simulink model "PID"  (R2024b)
settings: Solver=FixedStepAuto  StartTime=0.0  StopTime=inf  FixedStep=0.001  RelTol=1e-3  EnableMultiTasking=on
libraries: slpidlib x1, px4Peripheralslib x1, px4Sensorslib x1
settings Model: SimulationMode=external  ExtModeTrigDuration=10  Creator=ArriGE66  LastModifiedBy=xippa
settings SolverCC: PositivePriorityOrder=on
settings OptimizationCC: EnhancedBackFolding=on  PassReuseOutputArgsAs=Individual arguments  ZeroExternalMemoryAtStartup=off  ZeroInternalMemoryAtStartup=off  MaxStackSize=64  OptimizeBlockOrder=speed  DifferentSizesBufferReuse=on  OptimizationCustomize=off  EfficientTunableParamExpr=on
settings DebuggingCC: ParameterTunabilityLossMsg=error
settings HardwareCC: ProdBitPerPointer=32  ProdBitPerSizeT=32  ProdBitPerPtrDiffT=32  ProdLargestAtomicInteger=Long  ProdLargestAtomicFloat=Double  ProdWordSize=32  ProdLongLongMode=on  ProdHWDeviceType=ARM Compatible->ARM Cortex
settings SFSimCC: MATLABDynamicMemAlloc=off  SimTargetLang=C++
settings RTWCC: Description=Embedded Coder  SystemTargetFile=ert.tlc  HardwareBoard=PX4 Cube Orange  TemplateMakefile=ert_default_tmf  Toolchain=GNU Tools for PX4 Autopilots  TargetLang=C++  GPUComputeCapability=3.5
settings CodeAppCC: ForceParamTrailComments=on  IgnoreCustomStorageClasses=off  OperatorAnnotations=on  SimulinkDataObjDesc=on  SFDataObjDesc=on  InsertBlockDesc=on
settings ERTTargetCC: SupportVariableSizeSignals=on  ExtMode=on  ExtModeTransport=3  ExtModeStaticAlloc=on  ExtModeStaticAllocSize=1024  ExtModeMexFile=ext_xcp  ExtModeMexArgs=1 COM10 3000000  ExtModeIntrfLevel=Level2 - Open  InlinedParameterPlacement=Hierarchical  DynamicArrayContainerType=coder::array

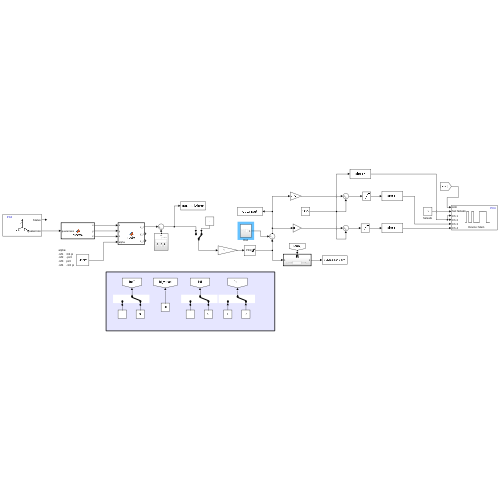
[thumbnail: Simulink's stored preview of the top-level diagram]
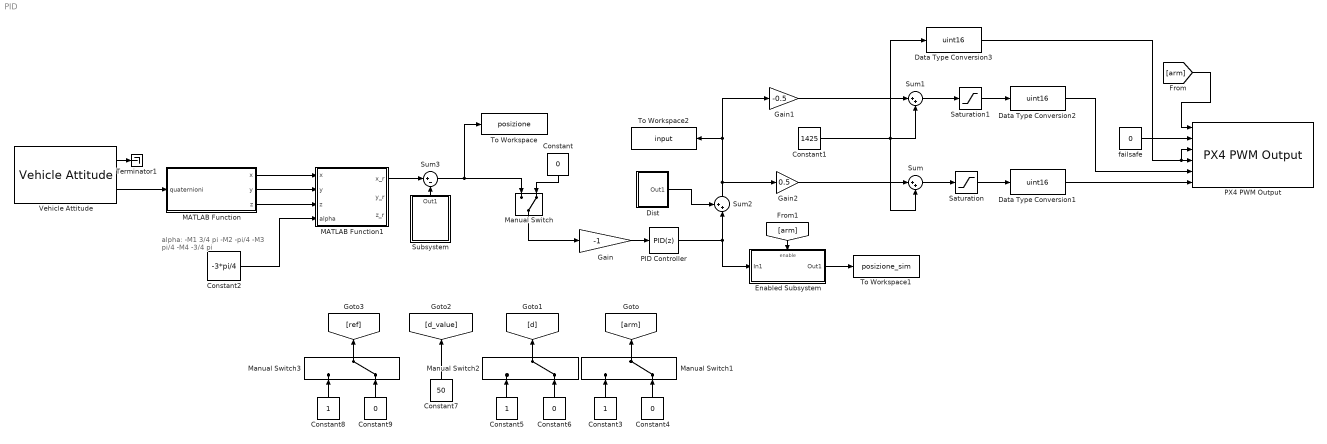
== system PID ==
  note: alpha:
      | -M1    3/4 pi
      | -M2    -pi/4
      | -M3    pi/4
      | -M4    -3/4 pi
  Constant{,4,6,9} (4 alike) : Constant  Value=0
  Constant1 : Constant  Value=1425  SampleTime=0.01
  Constant2 : Constant  Value=-3*pi/4  SampleTime=0.01
  Constant3 : Constant
  Constant5 : Constant
  Constant7 : Constant  Value=50
  Constant8 : Constant
  Data Type Conversion1 : DataTypeConversion  OutDataTypeStr=uint16  SaturateOnIntegerOverflow=off  RndMeth=Floor
  Data Type Conversion2 : DataTypeConversion  OutDataTypeStr=uint16  SaturateOnIntegerOverflow=off  RndMeth=Floor
  Data Type Conversion3 : DataTypeConversion  OutDataTypeStr=uint16  SaturateOnIntegerOverflow=off  RndMeth=Floor
  Dist : Subsystem
  Enabled Subsystem : Subsystem  TreatAsAtomicUnit=on
  Gain : Gain  Gain=-1
  Gain1 : Gain  Gain=-0.5
  Gain2 : Gain  Gain=0.5
  MATLAB Function : MATLAB Function  TreatAsAtomicUnit=on
  MATLAB Function1 : MATLAB Function  TreatAsAtomicUnit=on
  Manual Switch{,1..3} (4 alike) : ManualSwitch  CurrentSetting=0
  PID Controller : slpidlib/PID Controller  Controller=PID  Form=Parallel  TimeDomain=Discrete-time  UseExternalTs=off  SampleTime=-1  IntegratorMethod=Forward Euler  FilterMethod=Forward Euler  ControllerParametersSource=internal  P=400  I=500  UseKiTs=off  D=50  UseExternalDerivativeSource=off  N=880  UseFilter=on  TunerSelectOption=Transfer Function Based (PID Tuner App)  InitialConditionSource=internal  InitialConditionForIntegrator=0  InitialConditionForFilter=0  DifferentiatorICPrevScaledInput=0  ExternalReset=none  TrackingMode=off  Kt=1  LimitOutput=on  SatLimitsSource=internal  UpperSaturationLimit=600  LowerSaturationLimit=-600  LinearizeAsGain=on  AntiWindupMode=clamping  Kb=1  LimitIntegrator=off  UpperIntegratorSaturationLimit=inf  LowerIntegratorSaturationLimit=-inf  POutMin=[]  POutMax=[]  IOutMin=[]  IOutMax=[]  DOutMin=[]  DOutMax=[]  NOutMin=[]  NOutMax=[]  SumOutMin=[]  SumOutMax=[]  SaturationOutMin=[]  SaturationOutMax=[]  PParamMin=[]  PParamMax=[]  IParamMin=[]  IParamMax=[]  DParamMin=[]  DParamMax=[]  NParamMin=[]  NParamMax=[]  KbParamMin=[]  KbParamMax=[]  KtParamMin=[]  KtParamMax=[]  KbOutMin=[]  KbOutMax=[]  KtOutMin=[]  KtOutMax=[]  IntegratorOutMin=[]  IntegratorOutMax=[]  FilterOutMin=[]  FilterOutMax=[]  SumI1OutMin=[]  SumI1OutMax=[]  SumI2OutMin=[]  SumI2OutMax=[]  SumI3OutMin=[]  SumI3OutMax=[]  SumI4OutMin=[]  SumI4OutMax=[]  SumDOutMin=[]  SumDOutMax=[]  DifferentiatorOutMin=[]  DifferentiatorOutMax=[]  FilterDiffOutCoefMin=[]  FilterDiffOutCoefMax=[]  ReciprocalOutMin=[]  ReciprocalOutMax=[]  SumDenOutMin=[]  SumDenOutMax=[]  SumNumOutMin=[]  SumNumOutMax=[]  DivideOutMin=[]  DivideOutMax=[]  UdiffTsProdOutMin=[]  UdiffTsProdOutMax=[]  NTsProdOutMin=[]  NTsProdOutMax=[]  UintegralTsProdOutMin=[]  UintegralTsProdOutMax=[]  UngainTsProdOutMin=[]  UngainTsProdOutMax=[]  ClampingZeroOutDataTypeStr=Inherit: Inherit via back propagation  ClampingZeroOutMin=[]  ClampingZeroOutMax=[]  FilterDenConstantOutDataTypeStr=Inherit: Inherit via back propagation  FilterDenConstantOutMin=[]  FilterDenConstantOutMax=[]  PCopyOutDataTypeStr=Inherit: Inherit via back propagation  PCopyOutMin=[]  PCopyOutMax=[]  NCopyOutDataTypeStr=Inherit: Inherit via back propagation  NCopyOutMin=[]  NCopyOutMax=[]  IntegratorContinuousStateAttributes=''  IntegratorStateMustResolveToSignalObject=off  IntegratorRTWStateStorageClass=Auto  FilterContinuousStateAttributes=''  FilterStateMustResolveToSignalObject=off  FilterRTWStateStorageClass=Auto  ParallelPVariant=InternalParameters  IdealPVariant=Disabled  IVariant=InternalParameters  DVariant=InternalParameters  IntegratorVariant=Discrete  SatVariant=Enabled  AWVariant=DiscClampingParallel  PCopyVariant=Disabled  TRVariant=Disabled  FdbkBlocksVariant=Forward  IdealPFdbkVariant=Disabled  SatFdbkVariant=Disabled  DerivativeFilterVariant=ForwardEulerFilter  NVariant=InternalParameters  NCopyVariant=Disabled  FilterICVariant=InternalICsFilter  IntegratorICVariant=InternalICs  ExternalResetVariant=Disabled  TRSumVariant=Passthrough  SumFdbkVariant=Disabled  SumVariant=Sum_PID  TsampFilterVariant=InternalTs  TsampNgainVariant=Passthrough  TsampIntegralVariant=Disabled_SignalSpec  ExternalSaturationOutDataTypeStr=Inherit: Same as second input  DerivativeSourceVariant=ErrorSignal  PreIntVariant=InternalPreInt
  PX4 PWM Output : px4Peripheralslib/PX4 PWM Output  pwmDevice=Main  pwmChannel1_=on  pwmChannel2_=on  pwmChannel3_=on  pwmChannel4_=on  pwmChannel5_=off  pwmChannel6_=off  pwmChannel7_=off  pwmChannel8_=off
  Saturation : Saturate  UpperLimit=1750  LowerLimit=1050
  Saturation1 : Saturate  UpperLimit=1750  LowerLimit=1050
  Subsystem : Subsystem
  Sum : Sum  Inputs=|++
  Sum1 : Sum  Inputs=|++
  Sum2 : Sum  Inputs=++|
  Sum3 : Sum  Inputs=|+-
  Terminator1 : Terminator
  To Workspace : ToWorkspace  VariableName=posizione  SaveFormat=Timeseries  SampleTime=-1
  To Workspace1 : ToWorkspace  VariableName=posizione_sim  SaveFormat=Timeseries  SampleTime=-1
  To Workspace2 : ToWorkspace  VariableName=input  SaveFormat=Timeseries  SampleTime=-1
  Vehicle Attitude : px4Sensorslib/Vehicle Attitude  rollRate=off  pitchRate=off  yawRate=off  quaternion=on  uorbTimeStamp=off  BlockingMode=off  BlockTimeout=0.001  sampleTime=0.01
  failsafe : Constant  Value=0  OutDataTypeStr=boolean  SampleTime=0.01
  wires:
  Gain1/1 -> Sum1/1
  Data Type Conversion2/1 -> PX4 PWM Output/5
  Sum/1 -> Saturation/1
  Gain2/1 -> Sum/1
  MATLAB Function/2(y) -> MATLAB Function1/2(y)
  MATLAB Function/1(x) -> MATLAB Function1/1(x)
  MATLAB Function/3(z) -> MATLAB Function1/3(z)
  Constant1/1 -> Sum1/2, Data Type Conversion3/1, Sum/2
  Data Type Conversion1/1 -> PX4 PWM Output/6
  failsafe/1 -> PX4 PWM Output/2
  Sum1/1 -> Saturation1/1
  Vehicle Attitude/2 -> MATLAB Function/1(quaternioni)
  Data Type Conversion3/1 -> PX4 PWM Output/3, PX4 PWM Output/4
  PID Controller/1 -> Sum2/2, Enabled Subsystem/1(In1)
  Constant2/1 -> MATLAB Function1/4(alpha)
  Vehicle Attitude/1 -> Terminator1/1
  Gain/1 -> PID Controller/1
  Manual Switch/1 -> Gain/1
  Saturation/1 -> Data Type Conversion1/1
  Saturation1/1 -> Data Type Conversion2/1
  Constant/1 -> Manual Switch/2
  [arm] -> PX4 PWM Output/1
  Manual Switch1/1 -> [arm]
  Constant4/1 -> Manual Switch1/2
  Constant3/1 -> Manual Switch1/1
  [arm] -> Enabled Subsystem/Enable
  Enabled Subsystem/1(Out1) -> To Workspace1/1
  Sum2/1 -> To Workspace2/1, Gain1/1, Gain2/1
  Dist/1(Out1) -> Sum2/1
  Constant5/1 -> Manual Switch2/1
  Constant6/1 -> Manual Switch2/2
  Manual Switch2/1 -> [d]
  Constant7/1 -> [d_value]
  MATLAB Function1/1(x_r) -> Sum3/1
  Sum3/1 -> Manual Switch/1, To Workspace/1
  Subsystem/1(Out1) -> Sum3/2
  Constant8/1 -> Manual Switch3/1
  Manual Switch3/1 -> [ref]
  Constant9/1 -> Manual Switch3/2

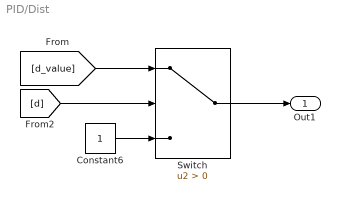
== system PID/Dist ==
  Constant6 : Constant
  Switch : Switch  Criteria=u2 > Threshold  SaturateOnIntegerOverflow=off  InputSameDT=off
  Out1 : Outport
  wires:
  [d] -> Switch/2
  Constant6/1 -> Switch/3
  Switch/1 -> Out1/1
  [d_value] -> Switch/1

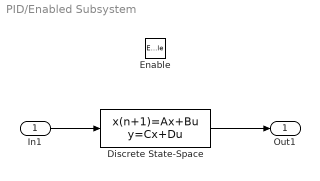
== system PID/Enabled Subsystem ==
  In1 : Inport
  Enable : EnablePort
  Discrete State-Space : DiscreteStateSpace  SampleTime=-1
  Out1 : Outport
  wires:
  Discrete State-Space/1 -> Out1/1
  In1/1 -> Discrete State-Space/1

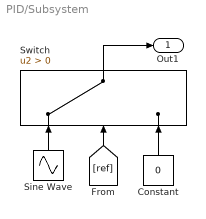
== system PID/Subsystem ==
  Constant : Constant  Value=0
  Sine Wave : Sin  Amplitude=0.1  SampleTime=0
  Switch : Switch  Criteria=u2 > Threshold  SaturateOnIntegerOverflow=off  InputSameDT=off
  Out1 : Outport
  wires:
  Switch/1 -> Out1/1
  [ref] -> Switch/2
  Sine Wave/1 -> Switch/1
  Constant/1 -> Switch/3

== matlab function PID/MATLAB Function1 ==
  data: x input; y input; z input; x_r output; alpha input; y_r output; z_r output
function [x_r,y_r,z_r] = ruoto(x,y,z,alpha)
Global_POV = [x y z];
R_z = [cos(alpha), -sin(alpha), 0;
       sin(alpha), cos(alpha), 0;
       0, 0, 1];
LOCALPOV = Global_POV * R_z;
x_r = LOCALPOV(1);
y_r = LOCALPOV(2);
z_r = LOCALPOV(3);
end

== matlab function PID/MATLAB Function ==
  data: x output; y output; quaternioni input; z output
function [x, y, z] = assetto(quaternioni)
    % Estrazione dei componenti del quaternione
    qw = quaternioni(1);
    qx = quaternioni(2);
    qy = quaternioni(3);
    qz = quaternioni(4);

    % Calcolo degli angoli di Eulero manualmente
    x = atan2(2*(qw*qx + qy*qz), 1 - 2*(qx^2 + qy^2)); % roll
    y = asin(2*(qw*qy - qz*qx));                          % Pitch
    z = atan2(2*(qw*qz + qx*qy), 1 - 2*(qy^2 + qz^2));   % yaw
end
